simulink model "m3dscope_new"  (Simulink 8.4)
settings: Solver=FixedStepDiscrete  StartTime=0.0  StopTime=10.0  RelTol=1e-3
undefined symbols (not defined in the file or in its folder): sfun3d
settings Model: Creator=gcampa  LastModifiedBy=gcampa  CovModelRefEnable=off  CovSFcnEnable=on
settings DataIOCC: SaveFormat=StructureWithTime  SignalLoggingSaveFormat=Dataset
settings OptimizationCC: ExpressionDepthLimit=128
settings DebuggingCC: UnderspecifiedInitializationDetection=Simplified  MergeDetectMultiDrivingBlocksExec=error  SolverPrmCheckMsg=none  FcnCallInpInsideContextMsg=EnableAllAsError  FrameProcessingCompatibilityMsg=error  StateNameClashWarn=none
settings HardwareCC: ProdBitPerPointer=64  ProdLargestAtomicFloat=Float  ProdIntDivRoundTo=Zero  ProdEndianess=LittleEndian  ProdHWDeviceType=Specified
settings GRTTargetCC: GeneratePreprocessorConditionals=Use local settings  CombineOutputUpdateFcns=on  GRTInterface=off

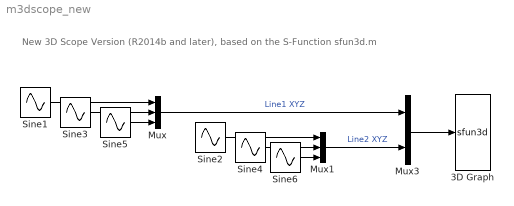
== system m3dscope_new ==
  note: New 3D Scope Version (R2014b and later), based on the S-Function sfun3d.m
  3D Graph : S-Function  LoadFcn=sfun3d([],[],[],'LoadBlock')  StartFcn=sfun3d([],[],[],'Start')  StopFcn=sfun3d([],[],[],'Stop')  FunctionName=sfun3d  Parameters=ax,T,np,cp,gd,ls,mk  EnableBusSupport=off  mask(3D Graph){np=2, ax=[-3 3 -3 3 -3 3], cp=[3 2 1], gd=on, ls=-, mk=none, T=0.1}
      mask prompts: np "Number of point (lines)"; ax "[xmin xmax  ymin ymax zmin zmax]"; cp "Camera position (use [0 0 1] for 2D XY view)"; gd "Grid (on|off)"; ls "LineStyle"; mk "Marker"; T "Sampling Time"
      mask help:
      | This block plots the position of several points in the XYZ space. The input contains the coordinates of all the points (x1,y1,z1,x2,y2,z2,...).
      | The number of points (lines), the XYZ ranges, camera position, grid, linestyle, marker and sampling time, can be set as mask parameters.
      settings: CopyFcn=sfun3d([],[],[],'CopyBlock')  DeleteFcn=sfun3d([],[],[],'DeleteBlock')  NameChangeFcn=sfun3d([],[],[],'NameChange')
      mask Help:
      | This block plots the position of several points in the XYZ space. The input contains the coordinates of all the points (x1,y1,z1,x2,y2,z2,...).
      | The number of points (lines), the XYZ ranges, camera position, grid, linestyle, marker and sampling time, can be set as mask parameters.
      mask TypeOptions ls: - | -- | : | -. | none
      mask TypeOptions mk: none | . | + | o | * | x | square | diamond | v | ^ | > | < | pentagram | hexagram
      mask Display: plot([.05 .95 .95 .05 .05],[.45 .45 .95 .95 .45], 0.5+cos(0:0.1:2*pi)*0.3,0.7+sin(0:0.1:2*pi)*0.2)
  Mux : Mux  Inputs=3
  Mux1 : Mux  Inputs=3
  Mux3 : Mux  Inputs=2
  Sine1 : Sin  SampleTime=0
  Sine2 : Sin  Amplitude=2  Frequency=2  SampleTime=0
  Sine3 : Sin  Phase=pi/2  SampleTime=0
  Sine4 : Sin  Amplitude=2  Frequency=2  Phase=pi/2  SampleTime=0
  Sine5 : Sin  Amplitude=1.5  Frequency=1.2  Phase=pi/2  SampleTime=0
  Sine6 : Sin  Amplitude=2.5  Frequency=2.2  Phase=pi/2  SampleTime=0
  wires:
  Mux/1 -> Mux3/1  "Line1 XYZ"
  Sine1/1 -> Mux/1
  Sine3/1 -> Mux/2
  Sine5/1 -> Mux/3
  Mux1/1 -> Mux3/2  "Line2 XYZ"
  Sine2/1 -> Mux1/1
  Sine6/1 -> Mux1/3
  Sine4/1 -> Mux1/2
  Mux3/1 -> 3D Graph/1
